simulink model "reference"  (R2024b)
settings: Solver=ode4  StartTime=0.0  StopTime=500  FixedStep=0.01  RelTol=1e-3
values from neighbouring files (symbols this model uses):
  aeroData = evalin('base','aeroData')    [CostTrim.m]    (also in aeroData_HGDGUO.mat = )
  b = evalin('base','b')    [CostTrim.m]    (also in UnmannedAerialVehicle.m = 10)
  cbar = evalin('base','cbar')    [CostTrim.m]    (also in UnmannedAerialVehicle.m = 1.32)
  CG = evalin('base','CG')    [CostTrim.m]    (also in UnmannedAerialVehicle.m = [0 0 0])
  CP = evalin('base','CP')    [CostTrim.m]    (also in UnmannedAerialVehicle.m = [3693.677 10.138 28.311]*1e-3)
  force_p1 = evalin('base','force_p1')    [CostTrim.m]    (also in UnmannedAerialVehicle.m = 2347)
  force_p2 = evalin('base','force_p2')    [CostTrim.m]    (also in UnmannedAerialVehicle.m = -32.38)
  Mass = evalin('base','Mass')    [CostTrim.m]    (also in UAVProperty.m = 600; UnmannedAerialVehicle.m = 600)
  S = evalin('base','S')    [CostTrim.m]    (also in UnmannedAerialVehicle.m = 13.2)
  torque_p1 = evalin('base','torque_p1')    [CostTrim.m]    (also in UnmannedAerialVehicle.m = 325.9)
  torque_p2 = evalin('base','torque_p2')    [CostTrim.m]    (also in UnmannedAerialVehicle.m = -5.774)
libraries: aerolibasang x2, simulink_extras x2, shared6dof x1, matrix_library x1, aerolibtransform2 x1, aerolibatmos2 x1
settings Model: Creator=LocoalKOH  LastModifiedBy=LocoalKOH

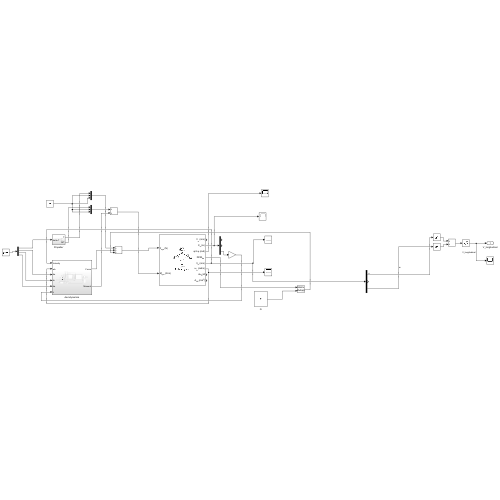
[thumbnail: Simulink's stored preview of the top-level diagram]
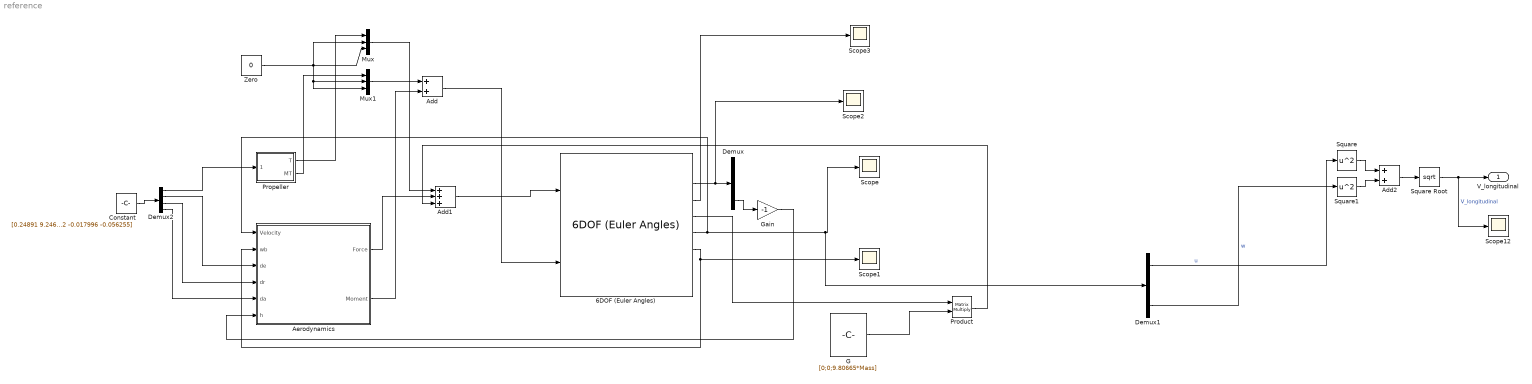
== system reference ==
  6DOF (Euler Angles) : shared6dof/6DOF (Euler Angles)  units=Metric (MKS)  mtype=Fixed  rep=Euler Angles  xme_0=[6.7306e-16 0 -500]  Vm_0=[39.959 0 1.8114]  eul_0=[-0.00017997 0.0453 -8.1523e-06]  pm_0=[1.5809e-18 -2.7281e-19 -3.1299e-19]  mass_0=Mass  mass_e=0.5  mass_f=2.0  inertia=I  inertia_e=eye(3)  inertia_f=2*eye(3)  k_quat=1.0  vre_flag=on  abi_flag=off  aMode=0  xme_statename=''  Vm_statename=''  eul_statename=''  quat_statename=''  pm_statename=''  mass_statename=''
  Add : Sum
  Add1 : Sum  Inputs=+++
  Add2 : Sum
  Aerodynamics : Subsystem
  Constant : Constant  Value=[0.24891 9.2462 -0.017996 -0.056255]
  Demux : Demux  Outputs=3
  Demux1 : Demux  Outputs=3
  Demux2 : Demux
  G : Constant  Value=[0;0;9.80665*Mass]  VectorParams1D=off
  Gain : Gain  Gain=-1
  Mux : Mux  Inputs=3
  Mux1 : Mux  Inputs=3
  Product : Product  Multiplication=Matrix(*)
  Propeller : Subsystem
  Scope{,1..3,12} (5 alike) : Scope
  Square : Math  Operator=square
  Square Root : Sqrt
  Square1 : Math  Operator=square
  Zero : Constant  Value=0  OutDataTypeStr=Inherit: Inherit via back propagation
  V_longitudinal : Outport
  wires:
  6DOF (Euler Angles)/5 -> Demux1/1, Scope/1, Aerodynamics/1(Velocity)
  6DOF (Euler Angles)/6 -> Scope1/1, Aerodynamics/2(wb)
  6DOF (Euler Angles)/2 -> Scope2/1, Demux/1
  Demux/3 -> Gain/1
  Gain/1 -> Aerodynamics/6(h)
  Zero/1 -> Mux1/3, Mux1/2, Mux/3, Mux/2
  Propeller/1(T) -> Mux/1
  Propeller/2(MT) -> Mux1/1
  Mux1/1 -> Add/1
  Aerodynamics/2(Moment) -> Add/2
  Add/1 -> 6DOF (Euler Angles)/2
  Mux/1 -> Add1/1
  Aerodynamics/1(Force) -> Add1/2
  Add1/1 -> 6DOF (Euler Angles)/1
  6DOF (Euler Angles)/3 -> Scope3/1
  Product/1 -> Add1/3
  G/1 -> Product/2
  6DOF (Euler Angles)/4 -> Product/1
  Demux1/3 -> Square1/1  "w"
  Square Root/1 -> Scope12/1, V_longitudinal/1  "V_longitudinal"
  Demux1/1 -> Square/1  "u"
  Square/1 -> Add2/1
  Add2/1 -> Square Root/1
  Square1/1 -> Add2/2
  Constant/1 -> Demux2/1
  Demux2/1 -> Propeller/1(delta T)
  Demux2/2 -> Aerodynamics/3(de)
  Demux2/3 -> Aerodynamics/4(dr)
  Demux2/4 -> Aerodynamics/5(da)

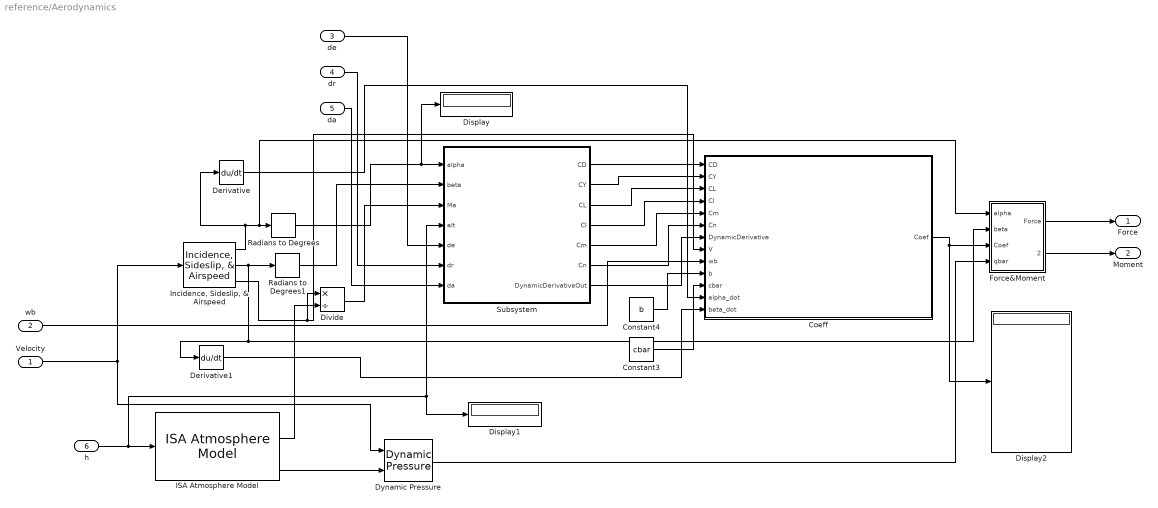
== system reference/Aerodynamics ==
  Velocity : Inport
  wb : Inport  Port=2
  de : Inport  Port=3
  dr : Inport  Port=4
  da : Inport  Port=5
  h : Inport  Port=6
  Coeff : MATLAB Function  TreatAsAtomicUnit=on
  Constant3 : Constant  Value=cbar
  Constant4 : Constant  Value=b
  Derivative : Derivative
  Derivative1 : Derivative
  Display : Display
  Display1 : Display
  Display2 : Display
  Divide : Product  Inputs=*/
  Dynamic Pressure : aerolibasang/Dynamic Pressure
  Force&Moment : Subsystem
  ISA Atmosphere Model : aerolibatmos2/ISA Atmosphere Model  useExtended=off  action=Warning  custom=off  viscosityOut=off  g=9.80665  gamma=1.4  R=287.0531  L=0.0065  h_trop=11000  h_strat=20000  rho0=1.225  P0=101325  T0=288.15  h0=0  S=110.4  Tref=273.15  muref=1.716e-5
  "Incidence, Sideslip, & Airspeed" : aerolibasang/Incidence, Sideslip, & Airspeed
  Radians to Degrees : simulink_extras/Transformations/Radians to Degrees
  Radians to Degrees1 : simulink_extras/Transformations/Radians to Degrees
  Subsystem : Subsystem
  Force : Outport
  Moment : Outport  Port=2
  wires:
  "Incidence, Sideslip, & Airspeed"/1 -> Derivative/1, Force&Moment/1(alpha), Radians to Degrees/1
  "Incidence, Sideslip, & Airspeed"/2 -> Force&Moment/2(beta), Derivative1/1, Radians to Degrees1/1
  h/1 -> Subsystem/4(alt), Display1/1, ISA Atmosphere Model/1
  ISA Atmosphere Model/4 -> Dynamic Pressure/2
  Dynamic Pressure/1 -> Force&Moment/4(qbar)
  Velocity/1 -> Dynamic Pressure/1, "Incidence, Sideslip, & Airspeed"/1
  Force&Moment/1(Force) -> Force/1
  Force&Moment/2(Moment) -> Moment/1
  Subsystem/1(CD) -> Coeff/1(CD)
  Subsystem/2(CY) -> Coeff/2(CY)
  Subsystem/3(CL) -> Coeff/3(CL)
  Subsystem/4(Cl) -> Coeff/4(Cl)
  Subsystem/5(Cm) -> Coeff/5(Cm)
  Subsystem/6(Cn) -> Coeff/6(Cn)
  Subsystem/7(DynamicDerivativeOut) -> Coeff/7(DynamicDerivative)
  Coeff/1(Coef) -> Display2/1, Force&Moment/3(Coef)
  Constant4/1 -> Coeff/10(b)
  Constant3/1 -> Coeff/11(cbar)
  Derivative/1 -> Coeff/12(alpha_dot)
  Derivative1/1 -> Coeff/13(beta_dot)
  "Incidence, Sideslip, & Airspeed"/3 -> Divide/1, Coeff/8(V)
  wb/1 -> Coeff/9(wb)
  Radians to Degrees/1 -> Display/1, Subsystem/1(alpha)
  Radians to Degrees1/1 -> Subsystem/2(beta)
  de/1 -> Subsystem/5(de)
  dr/1 -> Subsystem/6(dr)
  da/1 -> Subsystem/7(da)
  Divide/1 -> Subsystem/3(Ma)
  ISA Atmosphere Model/2 -> Divide/2

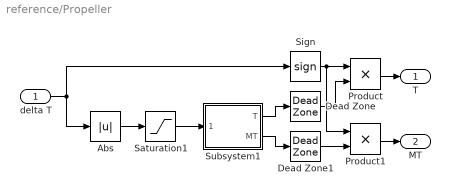
== system reference/Propeller ==
  delta T : Inport
  Abs : Abs  SaturateOnIntegerOverflow=off
  Dead Zone : DeadZone  LowerValue=-Inf  UpperValue=0
  Dead Zone1 : DeadZone  LowerValue=-Inf  UpperValue=0
  Product : Product
  Product1 : Product
  Saturation1 : Saturate  UpperLimit=0.85  LowerLimit=0
  Sign : Signum
  Subsystem1 : Subsystem
  T : Outport
  MT : Outport  Port=2
  wires:
  Saturation1/1 -> Subsystem1/1(delta T)
  Subsystem1/2(MT) -> Dead Zone1/1
  delta T/1 -> Abs/1, Sign/1
  Dead Zone1/1 -> Product1/2
  Abs/1 -> Saturation1/1
  Dead Zone/1 -> Product/2
  Sign/1 -> Product1/1, Product/1
  Subsystem1/1(T) -> Dead Zone/1
  Product1/1 -> MT/1
  Product/1 -> T/1

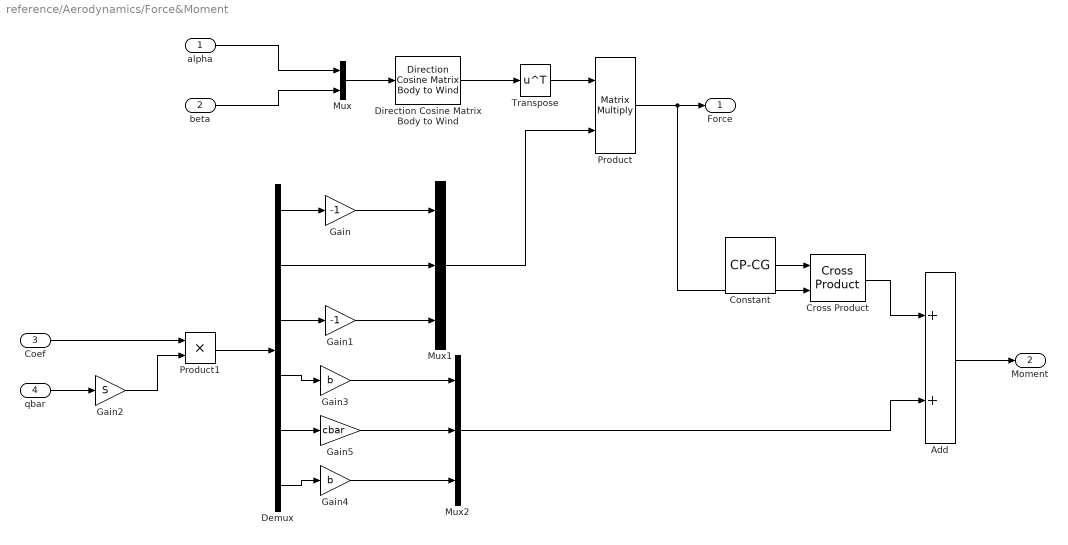
== system reference/Aerodynamics/Force&Moment ==
  alpha : Inport
  beta : Inport  Port=2
  Coef : Inport  Port=3
  qbar : Inport  Port=4
  Add : Sum
  Constant : Constant  Value=CP-CG  VectorParams1D=off
  Cross Product : matrix_library/Cross Product
  Demux : Demux  Outputs=6
  Direction Cosine Matrix Body to Wind : aerolibtransform2/Direction Cosine Matrix Body to Wind
  Gain : Gain  Gain=-1
  Gain1 : Gain  Gain=-1
  Gain2 : Gain  Gain=S
  Gain3 : Gain  Gain=b
  Gain4 : Gain  Gain=b
  Gain5 : Gain  Gain=cbar
  Mux : Mux  Inputs=2
  Mux1 : Mux  Inputs=3
  Mux2 : Mux  Inputs=3
  Product : Product  Multiplication=Matrix(*)
  Product1 : Product
  Transpose : Math  Operator=transpose
  Force : Outport
  Moment : Outport  Port=2
  wires:
  Coef/1 -> Product1/1
  Gain/1 -> Mux1/1
  Demux/6 -> Gain4/1
  Demux/3 -> Gain1/1
  Product/1 -> Force/1, Cross Product/2
  Transpose/1 -> Product/1
  Gain4/1 -> Mux2/3
  Demux/4 -> Gain3/1
  Gain5/1 -> Mux2/2
  Direction Cosine Matrix Body to Wind/1 -> Transpose/1
  Product1/1 -> Demux/1
  Mux2/1 -> Add/2
  Demux/2 -> Mux1/2
  Mux1/1 -> Product/2
  Cross Product/1 -> Add/1
  Demux/5 -> Gain5/1
  Constant/1 -> Cross Product/1
  Add/1 -> Moment/1
  Gain3/1 -> Mux2/1
  Demux/1 -> Gain/1
  Gain2/1 -> Product1/2
  qbar/1 -> Gain2/1
  Gain1/1 -> Mux1/3
  Mux/1 -> Direction Cosine Matrix Body to Wind/1
  beta/1 -> Mux/2
  alpha/1 -> Mux/1

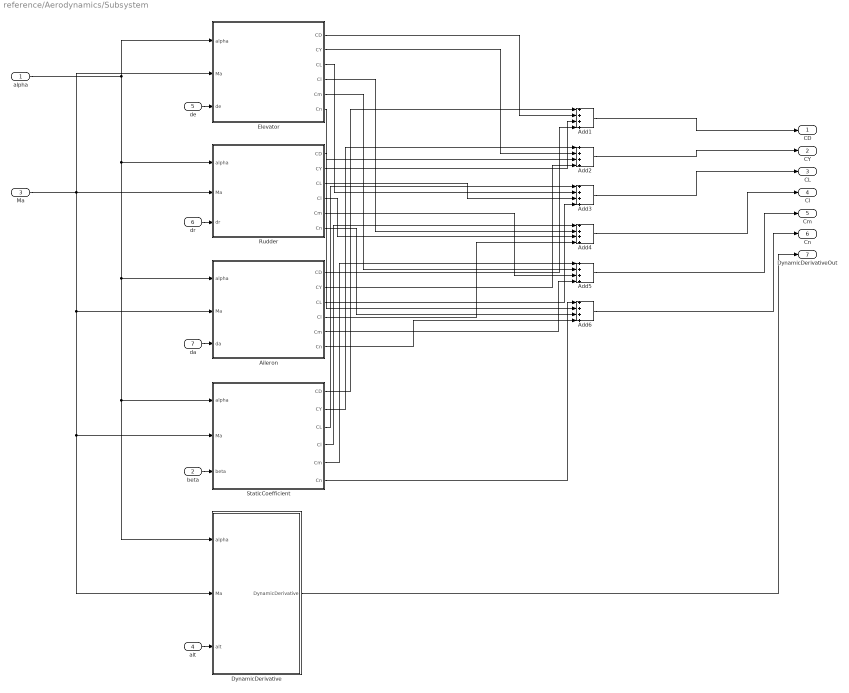
== system reference/Aerodynamics/Subsystem ==
  alpha : Inport
  beta : Inport  Port=2
  Ma : Inport  Port=3
  alt : Inport  Port=4
  de : Inport  Port=5
  dr : Inport  Port=6
  da : Inport  Port=7
  Add{1..6} (6 alike) : Sum  Inputs=++++
  Aileron : Subsystem
  DynamicDerivative : Subsystem
  Elevator : Subsystem
  Rudder : Subsystem
  StaticCoefficient : Subsystem
  CD : Outport
  CY : Outport  Port=2
  CL : Outport  Port=3
  Cl : Outport  Port=4
  Cm : Outport  Port=5
  Cn : Outport  Port=6
  DynamicDerivativeOut : Outport  Port=7
  wires:
  StaticCoefficient/4(Cl) -> Add4/1
  StaticCoefficient/2(CY) -> Add2/1
  Add3/1 -> CL/1
  Aileron/3(CL) -> Add3/4
  Aileron/1(CD) -> Add1/4
  Rudder/4(Cl) -> Add4/3
  de/1 -> Elevator/3(de)
  StaticCoefficient/3(CL) -> Add3/1
  da/1 -> Aileron/3(da)
  Elevator/2(CY) -> Add2/2
  dr/1 -> Rudder/3(dr)
  StaticCoefficient/6(Cn) -> Add6/1
  alt/1 -> DynamicDerivative/3(alt)
  Aileron/6(Cn) -> Add6/4
  beta/1 -> StaticCoefficient/3(beta)
  Elevator/3(CL) -> Add3/2
  Aileron/4(Cl) -> Add4/4
  StaticCoefficient/1(CD) -> Add1/1
  Elevator/5(Cm) -> Add5/2
  Aileron/5(Cm) -> Add5/4
  Elevator/6(Cn) -> Add6/2
  Rudder/5(Cm) -> Add5/3
  Elevator/1(CD) -> Add1/2
  StaticCoefficient/5(Cm) -> Add5/1
  Rudder/1(CD) -> Add1/3
  Rudder/6(Cn) -> Add6/3
  Rudder/2(CY) -> Add2/3
  Aileron/2(CY) -> Add2/4
  Ma/1 -> DynamicDerivative/2(Ma), StaticCoefficient/2(Ma), Aileron/2(Ma), Rudder/2(Ma), Elevator/2(Ma)
  Add2/1 -> CY/1
  Rudder/3(CL) -> Add3/3
  Elevator/4(Cl) -> Add4/2
  DynamicDerivative/1(DynamicDerivative) -> DynamicDerivativeOut/1
  Add4/1 -> Cl/1
  Add6/1 -> Cn/1
  Add1/1 -> CD/1
  Add5/1 -> Cm/1
  alpha/1 -> DynamicDerivative/1(alpha), StaticCoefficient/1(alpha), Aileron/1(alpha), Rudder/1(alpha), Elevator/1(alpha)

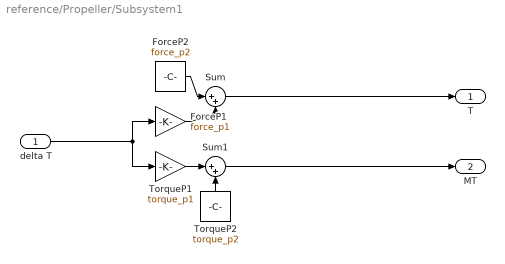
== system reference/Propeller/Subsystem1 ==
  delta T : Inport
  ForceP1 : Gain  Gain=force_p1
  ForceP2 : Constant  Value=force_p2
  Sum : Sum  Inputs=|++
  Sum1 : Sum  Inputs=|++
  TorqueP1 : Gain  Gain=torque_p1
  TorqueP2 : Constant  Value=torque_p2
  T : Outport
  MT : Outport  Port=2
  wires:
  Sum/1 -> T/1
  delta T/1 -> TorqueP1/1, ForceP1/1
  ForceP1/1 -> Sum/2
  Sum1/1 -> MT/1
  TorqueP1/1 -> Sum1/1
  ForceP2/1 -> Sum/1
  TorqueP2/1 -> Sum1/2

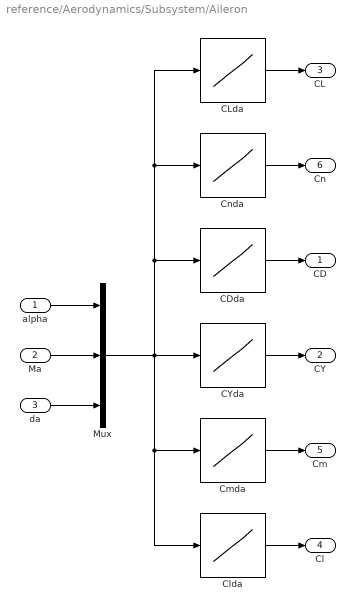
== system reference/Aerodynamics/Subsystem/Aileron ==
  alpha : Inport
  Ma : Inport  Port=2
  da : Inport  Port=3
  CDda : Lookup_n-D  NumberOfTableDimensions=3  LookupTableObject=test  BreakpointsForDimension1=aeroData.Vec_alpha  BreakpointsForDimension2=aeroData.Vec_Ma  BreakpointsForDimension3=[-15 0 15]  UseOneInputPortForAllInputData=on  Table=aeroData.CD_alpha_Ma_da  InternalRulePriority=Speed  RndMeth=Simplest
  CLda : Lookup_n-D  NumberOfTableDimensions=3  LookupTableObject=test  BreakpointsForDimension1=aeroData.Vec_alpha  BreakpointsForDimension2=aeroData.Vec_Ma  BreakpointsForDimension3=[-15 0 15]  UseOneInputPortForAllInputData=on  Table=aeroData.CL_alpha_Ma_da  InternalRulePriority=Speed  RndMeth=Simplest
  CYda : Lookup_n-D  NumberOfTableDimensions=3  LookupTableObject=test  BreakpointsForDimension1=aeroData.Vec_alpha  BreakpointsForDimension2=aeroData.Vec_Ma  BreakpointsForDimension3=[-15 0 15]  UseOneInputPortForAllInputData=on  Table=aeroData.CY_alpha_Ma_da  InternalRulePriority=Speed  RndMeth=Simplest
  Clda : Lookup_n-D  NumberOfTableDimensions=3  LookupTableObject=test  BreakpointsForDimension1=aeroData.Vec_alpha  BreakpointsForDimension2=aeroData.Vec_Ma  BreakpointsForDimension3=[-15 0 15]  UseOneInputPortForAllInputData=on  Table=aeroData.Cl_alpha_Ma_da  InternalRulePriority=Speed  RndMeth=Simplest
  Cmda : Lookup_n-D  NumberOfTableDimensions=3  LookupTableObject=test  BreakpointsForDimension1=aeroData.Vec_alpha  BreakpointsForDimension2=aeroData.Vec_Ma  BreakpointsForDimension3=[-15 0 15]  UseOneInputPortForAllInputData=on  Table=aeroData.Cm_alpha_Ma_da  InternalRulePriority=Speed  RndMeth=Simplest
  Cnda : Lookup_n-D  NumberOfTableDimensions=3  LookupTableObject=test  BreakpointsForDimension1=aeroData.Vec_alpha  BreakpointsForDimension2=aeroData.Vec_Ma  BreakpointsForDimension3=[-15 0 15]  UseOneInputPortForAllInputData=on  Table=aeroData.Cn_alpha_Ma_da  InternalRulePriority=Speed  RndMeth=Simplest
  Mux : Mux  Inputs=3
  CD : Outport
  CY : Outport  Port=2
  CL : Outport  Port=3
  Cl : Outport  Port=4
  Cm : Outport  Port=5
  Cn : Outport  Port=6
  wires:
  alpha/1 -> Mux/1
  Cnda/1 -> Cn/1
  Ma/1 -> Mux/2
  da/1 -> Mux/3
  Mux/1 -> CYda/1, Cmda/1, Clda/1, Cnda/1, CLda/1, CDda/1
  CDda/1 -> CD/1
  CLda/1 -> CL/1
  CYda/1 -> CY/1
  Cmda/1 -> Cm/1
  Clda/1 -> Cl/1

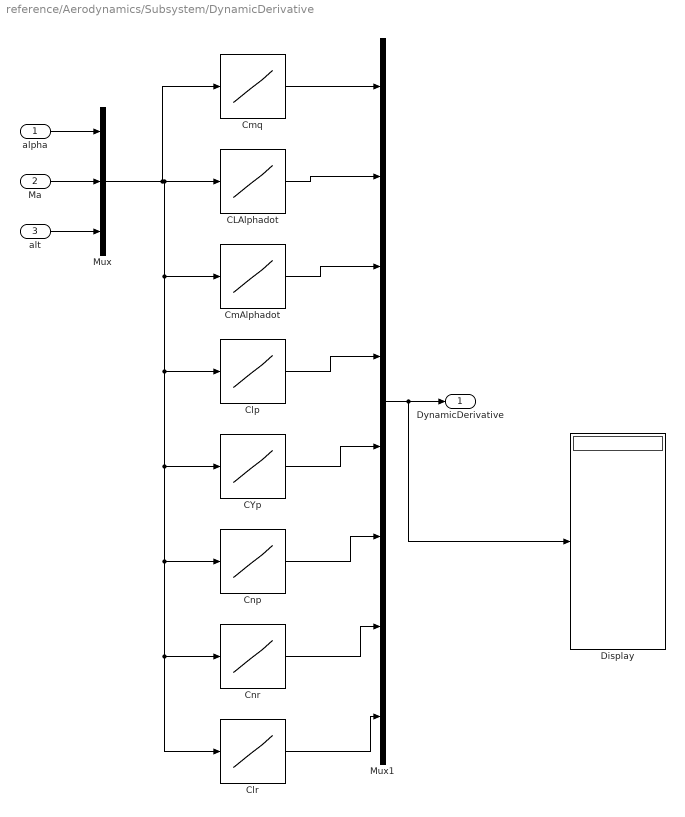
== system reference/Aerodynamics/Subsystem/DynamicDerivative ==
  alpha : Inport
  Ma : Inport  Port=2
  alt : Inport  Port=3
  CLAlphadot : Lookup_n-D  NumberOfTableDimensions=3  LookupTableObject=test  BreakpointsForDimension1=aeroData.Vec_alpha2  BreakpointsForDimension2=aeroData.Vec_Ma2  BreakpointsForDimension3=aeroData.Vec_alt  UseOneInputPortForAllInputData=on  Table=aeroData.CLAlphadot_alpha_Ma_alt  InternalRulePriority=Speed  RndMeth=Simplest
  CYp : Lookup_n-D  NumberOfTableDimensions=3  LookupTableObject=test  BreakpointsForDimension1=aeroData.Vec_alpha2  BreakpointsForDimension2=aeroData.Vec_Ma2  BreakpointsForDimension3=aeroData.Vec_alt  UseOneInputPortForAllInputData=on  Table=aeroData.CYp_alpha_Ma_alt  InternalRulePriority=Speed  RndMeth=Simplest
  Clp : Lookup_n-D  NumberOfTableDimensions=3  LookupTableObject=test  BreakpointsForDimension1=aeroData.Vec_alpha2  BreakpointsForDimension2=aeroData.Vec_Ma2  BreakpointsForDimension3=aeroData.Vec_alt  UseOneInputPortForAllInputData=on  Table=aeroData.Clp_alpha_Ma_alt  InternalRulePriority=Speed  RndMeth=Simplest
  Clr : Lookup_n-D  NumberOfTableDimensions=3  LookupTableObject=test  BreakpointsForDimension1=aeroData.Vec_alpha2  BreakpointsForDimension2=aeroData.Vec_Ma2  BreakpointsForDimension3=aeroData.Vec_alt  UseOneInputPortForAllInputData=on  Table=aeroData.Clr_alpha_Ma_alt  InternalRulePriority=Speed  RndMeth=Simplest
  CmAlphadot : Lookup_n-D  NumberOfTableDimensions=3  LookupTableObject=test  BreakpointsForDimension1=aeroData.Vec_alpha2  BreakpointsForDimension2=aeroData.Vec_Ma2  BreakpointsForDimension3=aeroData.Vec_alt  UseOneInputPortForAllInputData=on  Table=aeroData.CmAlphadot_alpha_Ma_alt  InternalRulePriority=Speed  RndMeth=Simplest
  Cmq : Lookup_n-D  NumberOfTableDimensions=3  LookupTableObject=test  BreakpointsForDimension1=aeroData.Vec_alpha2  BreakpointsForDimension2=aeroData.Vec_Ma2  BreakpointsForDimension3=aeroData.Vec_alt  UseOneInputPortForAllInputData=on  Table=aeroData.Cmq_alpha_Ma_alt  InternalRulePriority=Speed  RndMeth=Simplest
  Cnp : Lookup_n-D  NumberOfTableDimensions=3  LookupTableObject=test  BreakpointsForDimension1=aeroData.Vec_alpha2  BreakpointsForDimension2=aeroData.Vec_Ma2  BreakpointsForDimension3=aeroData.Vec_alt  UseOneInputPortForAllInputData=on  Table=aeroData.Cnp_alpha_Ma_alt  InternalRulePriority=Speed  RndMeth=Simplest
  Cnr : Lookup_n-D  NumberOfTableDimensions=3  LookupTableObject=test  BreakpointsForDimension1=aeroData.Vec_alpha2  BreakpointsForDimension2=aeroData.Vec_Ma2  BreakpointsForDimension3=aeroData.Vec_alt  UseOneInputPortForAllInputData=on  Table=aeroData.Cnr_alpha_Ma_alt  InternalRulePriority=Speed  RndMeth=Simplest
  Display : Display
  Mux : Mux  Inputs=3
  Mux1 : Mux  Inputs=8
  DynamicDerivative : Outport
  wires:
  alpha/1 -> Mux/1
  Ma/1 -> Mux/2
  Clp/1 -> Mux1/4
  alt/1 -> Mux/3
  Mux/1 -> Clr/1, Cnr/1, Cnp/1, CYp/1, Clp/1, CmAlphadot/1, CLAlphadot/1, Cmq/1
  CLAlphadot/1 -> Mux1/2
  Cmq/1 -> Mux1/1
  CmAlphadot/1 -> Mux1/3
  CYp/1 -> Mux1/5
  Cnp/1 -> Mux1/6
  Cnr/1 -> Mux1/7
  Clr/1 -> Mux1/8
  Mux1/1 -> Display/1, DynamicDerivative/1

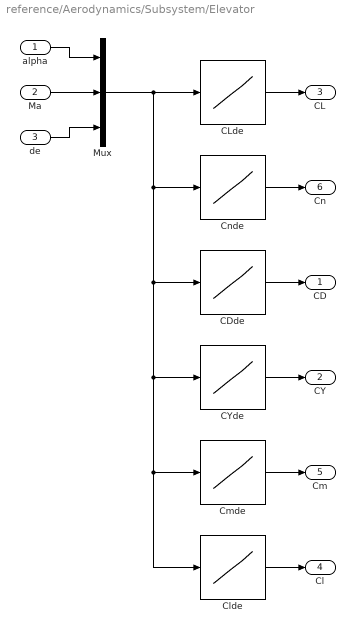
== system reference/Aerodynamics/Subsystem/Elevator ==
  alpha : Inport
  Ma : Inport  Port=2
  de : Inport  Port=3
  CDde : Lookup_n-D  NumberOfTableDimensions=3  LookupTableObject=test  BreakpointsForDimension1=aeroData.Vec_alpha  BreakpointsForDimension2=aeroData.Vec_Ma  BreakpointsForDimension3=[-15 0 15]  UseOneInputPortForAllInputData=on  Table=aeroData.CD_alpha_Ma_de  InternalRulePriority=Speed  RndMeth=Simplest
  CLde : Lookup_n-D  NumberOfTableDimensions=3  LookupTableObject=test  BreakpointsForDimension1=aeroData.Vec_alpha  BreakpointsForDimension2=aeroData.Vec_Ma  BreakpointsForDimension3=[-15 0 15]  UseOneInputPortForAllInputData=on  Table=aeroData.CL_alpha_Ma_de  InternalRulePriority=Speed  RndMeth=Simplest
  CYde : Lookup_n-D  NumberOfTableDimensions=3  LookupTableObject=test  BreakpointsForDimension1=aeroData.Vec_alpha  BreakpointsForDimension2=aeroData.Vec_Ma  BreakpointsForDimension3=[-15 0 15]  UseOneInputPortForAllInputData=on  Table=aeroData.CY_alpha_Ma_de  InternalRulePriority=Speed  RndMeth=Simplest
  Clde : Lookup_n-D  NumberOfTableDimensions=3  LookupTableObject=test  BreakpointsForDimension1=aeroData.Vec_alpha  BreakpointsForDimension2=aeroData.Vec_Ma  BreakpointsForDimension3=[-15 0 15]  UseOneInputPortForAllInputData=on  Table=aeroData.Cl_alpha_Ma_de  InternalRulePriority=Speed  RndMeth=Simplest
  Cmde : Lookup_n-D  NumberOfTableDimensions=3  LookupTableObject=test  BreakpointsForDimension1=aeroData.Vec_alpha  BreakpointsForDimension2=aeroData.Vec_Ma  BreakpointsForDimension3=[-15 0 15]  UseOneInputPortForAllInputData=on  Table=aeroData.Cm_alpha_Ma_de  InternalRulePriority=Speed  RndMeth=Simplest
  Cnde : Lookup_n-D  NumberOfTableDimensions=3  LookupTableObject=test  BreakpointsForDimension1=aeroData.Vec_alpha  BreakpointsForDimension2=aeroData.Vec_Ma  BreakpointsForDimension3=[-15 0 15]  UseOneInputPortForAllInputData=on  Table=aeroData.Cn_alpha_Ma_de  InternalRulePriority=Speed  RndMeth=Simplest
  Mux : Mux  Inputs=3
  CD : Outport
  CY : Outport  Port=2
  CL : Outport  Port=3
  Cl : Outport  Port=4
  Cm : Outport  Port=5
  Cn : Outport  Port=6
  wires:
  Cnde/1 -> Cn/1
  alpha/1 -> Mux/1
  Mux/1 -> Clde/1, Cmde/1, CYde/1, CDde/1, Cnde/1, CLde/1
  Ma/1 -> Mux/2
  de/1 -> Mux/3
  CYde/1 -> CY/1
  CDde/1 -> CD/1
  CLde/1 -> CL/1
  Cmde/1 -> Cm/1
  Clde/1 -> Cl/1

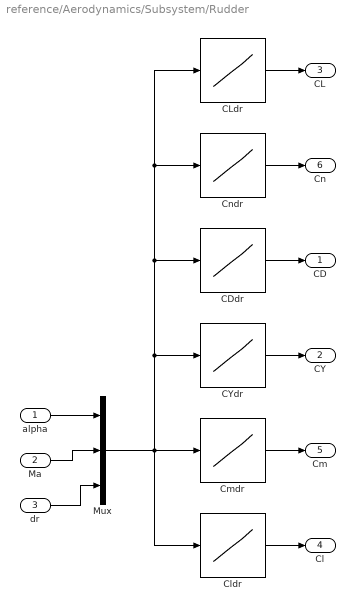
== system reference/Aerodynamics/Subsystem/Rudder ==
  alpha : Inport
  Ma : Inport  Port=2
  dr : Inport  Port=3
  CDdr : Lookup_n-D  NumberOfTableDimensions=3  LookupTableObject=test  BreakpointsForDimension1=aeroData.Vec_alpha  BreakpointsForDimension2=aeroData.Vec_Ma  BreakpointsForDimension3=[-15 0 15]  UseOneInputPortForAllInputData=on  Table=aeroData.CD_alpha_Ma_dr  InternalRulePriority=Speed  RndMeth=Simplest
  CLdr : Lookup_n-D  NumberOfTableDimensions=3  LookupTableObject=test  BreakpointsForDimension1=aeroData.Vec_alpha  BreakpointsForDimension2=aeroData.Vec_Ma  BreakpointsForDimension3=[-15 0 15]  UseOneInputPortForAllInputData=on  Table=aeroData.CL_alpha_Ma_dr  InternalRulePriority=Speed  RndMeth=Simplest
  CYdr : Lookup_n-D  NumberOfTableDimensions=3  LookupTableObject=test  BreakpointsForDimension1=aeroData.Vec_alpha  BreakpointsForDimension2=aeroData.Vec_Ma  BreakpointsForDimension3=[-15 0 15]  UseOneInputPortForAllInputData=on  Table=aeroData.CY_alpha_Ma_dr  InternalRulePriority=Speed  RndMeth=Simplest
  Cldr : Lookup_n-D  NumberOfTableDimensions=3  LookupTableObject=test  BreakpointsForDimension1=aeroData.Vec_alpha  BreakpointsForDimension2=aeroData.Vec_Ma  BreakpointsForDimension3=[-15 0 15]  UseOneInputPortForAllInputData=on  Table=aeroData.Cl_alpha_Ma_dr  InternalRulePriority=Speed  RndMeth=Simplest
  Cmdr : Lookup_n-D  NumberOfTableDimensions=3  LookupTableObject=test  BreakpointsForDimension1=aeroData.Vec_alpha  BreakpointsForDimension2=aeroData.Vec_Ma  BreakpointsForDimension3=[-15 0 15]  UseOneInputPortForAllInputData=on  Table=aeroData.Cm_alpha_Ma_dr  InternalRulePriority=Speed  RndMeth=Simplest
  Cndr : Lookup_n-D  NumberOfTableDimensions=3  LookupTableObject=test  BreakpointsForDimension1=aeroData.Vec_alpha  BreakpointsForDimension2=aeroData.Vec_Ma  BreakpointsForDimension3=[-15 0 15]  UseOneInputPortForAllInputData=on  Table=aeroData.Cn_alpha_Ma_dr  InternalRulePriority=Speed  RndMeth=Simplest
  Mux : Mux  Inputs=3
  CD : Outport
  CY : Outport  Port=2
  CL : Outport  Port=3
  Cl : Outport  Port=4
  Cm : Outport  Port=5
  Cn : Outport  Port=6
  wires:
  alpha/1 -> Mux/1
  CLdr/1 -> CL/1
  Mux/1 -> Cmdr/1, Cldr/1, Cndr/1, CLdr/1, CDdr/1, CYdr/1
  Ma/1 -> Mux/2
  Cldr/1 -> Cl/1
  dr/1 -> Mux/3
  Cndr/1 -> Cn/1
  CDdr/1 -> CD/1
  CYdr/1 -> CY/1
  Cmdr/1 -> Cm/1

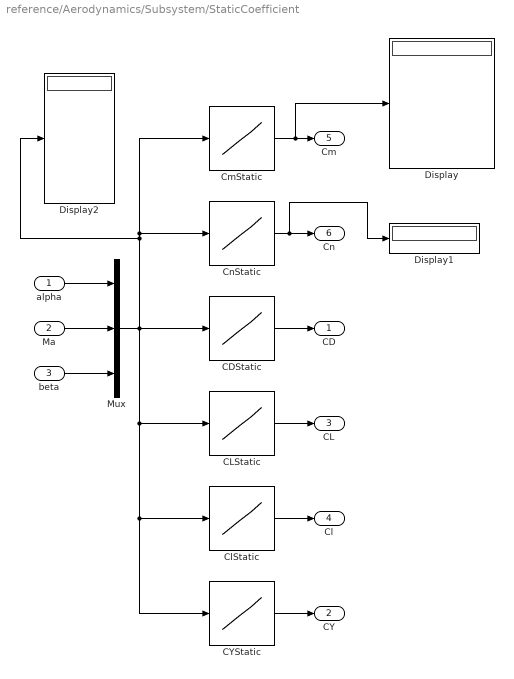
== system reference/Aerodynamics/Subsystem/StaticCoefficient ==
  alpha : Inport
  Ma : Inport  Port=2
  beta : Inport  Port=3
  CDStatic : Lookup_n-D  NumberOfTableDimensions=3  LookupTableObject=test  BreakpointsForDimension1=aeroData.Vec_alpha  BreakpointsForDimension2=aeroData.Vec_Ma  BreakpointsForDimension3=aeroData.Vec_beta  UseOneInputPortForAllInputData=on  Table=aeroData.CD_alpha_Ma_beta  InternalRulePriority=Speed  RndMeth=Simplest
  CLStatic : Lookup_n-D  NumberOfTableDimensions=3  LookupTableObject=test  BreakpointsForDimension1=aeroData.Vec_alpha  BreakpointsForDimension2=aeroData.Vec_Ma  BreakpointsForDimension3=aeroData.Vec_beta  UseOneInputPortForAllInputData=on  Table=aeroData.CL_alpha_Ma_beta  InternalRulePriority=Speed  RndMeth=Simplest
  CYStatic : Lookup_n-D  NumberOfTableDimensions=3  LookupTableObject=test  BreakpointsForDimension1=aeroData.Vec_alpha  BreakpointsForDimension2=aeroData.Vec_Ma  BreakpointsForDimension3=aeroData.Vec_beta  UseOneInputPortForAllInputData=on  Table=aeroData.CY_alpha_Ma_beta  InternalRulePriority=Speed  RndMeth=Simplest
  ClStatic : Lookup_n-D  NumberOfTableDimensions=3  LookupTableObject=test  BreakpointsForDimension1=aeroData.Vec_alpha  BreakpointsForDimension2=aeroData.Vec_Ma  BreakpointsForDimension3=aeroData.Vec_beta  UseOneInputPortForAllInputData=on  Table=aeroData.Cl_alpha_Ma_beta  InternalRulePriority=Speed  RndMeth=Simplest
  CmStatic : Lookup_n-D  NumberOfTableDimensions=3  LookupTableObject=test  BreakpointsForDimension1=aeroData.Vec_alpha  BreakpointsForDimension2=aeroData.Vec_Ma  BreakpointsForDimension3=aeroData.Vec_beta  UseOneInputPortForAllInputData=on  Table=aeroData.Cm_alpha_Ma_beta  InternalRulePriority=Speed  RndMeth=Simplest
  CnStatic : Lookup_n-D  NumberOfTableDimensions=3  LookupTableObject=test  BreakpointsForDimension1=aeroData.Vec_alpha  BreakpointsForDimension2=aeroData.Vec_Ma  BreakpointsForDimension3=aeroData.Vec_beta  UseOneInputPortForAllInputData=on  Table=aeroData.Cn_alpha_Ma_beta  InternalRulePriority=Speed  RndMeth=Simplest
  Display : Display
  Display1 : Display
  Display2 : Display
  Mux : Mux  Inputs=3
  CD : Outport
  CY : Outport  Port=2
  CL : Outport  Port=3
  Cl : Outport  Port=4
  Cm : Outport  Port=5
  Cn : Outport  Port=6
  wires:
  alpha/1 -> Mux/1
  CmStatic/1 -> Display/1, Cm/1
  Mux/1 -> CYStatic/1, ClStatic/1, CLStatic/1, Display2/1, CmStatic/1, CnStatic/1, CDStatic/1
  Ma/1 -> Mux/2
  beta/1 -> Mux/3
  CLStatic/1 -> CL/1
  CDStatic/1 -> CD/1
  CnStatic/1 -> Display1/1, Cn/1
  ClStatic/1 -> Cl/1
  CYStatic/1 -> CY/1

== matlab function reference/Aerodynamics/Coeff ==
  data: Coef output; CD input; CY input; CL input; Cl input; Cm input; Cn input; DynamicDerivative input; V input; wb input; b input; cbar input; alpha_dot input; beta_dot input
function Coef = CoefficientCalculator(CD,CY,CL,Cl,Cm,Cn,DynamicDerivative,V,wb,b,cbar,alpha_dot,beta_dot)
    p = wb(1);
    q = wb(2);
    r = wb(3);
    
    Cmq = DynamicDerivative(1);
    CLalphadot = DynamicDerivative(2);
    Cmalphadot = DynamicDerivative(3);
    Clp = DynamicDerivative(4);
    CYp = DynamicDerivative(5);
    Cnp = DynamicDerivative(6);
    Cnr = DynamicDerivative(7);
    Clr = DynamicDerivative(8);

    %没有的动导数数据写成0
    CDq = 0;
    CDalphadot = 0;
    CLq = 0;
    CYr = 0;
    Clbetadot = 0;
    Cnbetadot = 0;

    CD_dynamic = CDq*(q*cbar/(2*V)) + CDalphadot*(alpha_dot*cbar/(2*V));
    CL_dynamic = CLq*(q*cbar/(2*V)) + CLalphadot*(alpha_dot*cbar/(2*V));
    CY_dynamic = CYp*(p*b/(2*V)) + CYr*(r*b/(2*V));
    Cl_dynamic = Clp*(p*b/(2*V)) + Clr*(r*b/(2*V)) + Clbetadot*(beta_dot*b/(2*V));
    Cm_dynamic = Cmq*(q*cbar/(2*V)) + Cmalphadot*(alpha_dot*cbar/(2*V));
    Cn_dynamic = Cnp*(p*b/(2*V)) + Cnr*(r*b/(2*V)) + Cnbetadot*(beta_dot*b/(2*V));

    CD_sum = CD + CD_dynamic;
    CL_sum = CL + CL_dynamic;
    CY_sum = CY + CY_dynamic;
    Cl_sum = Cl + Cl_dynamic;
    Cm_sum = Cm + Cm_dynamic;
    Cn_sum = Cn + Cn_dynamic;

    Coef = [CD_sum; CY_sum; CL_sum; Cl_sum; Cm_sum; Cn_sum];
end
